simulink model "dc_motor_openloop_verification"  (R2026b)
settings: Solver=VariableStepAuto  StopTime=5.0
undefined symbols (not defined in the file): b, J, K, L, R
settings Model: Creator=nouran  LastModifiedBy=nouran

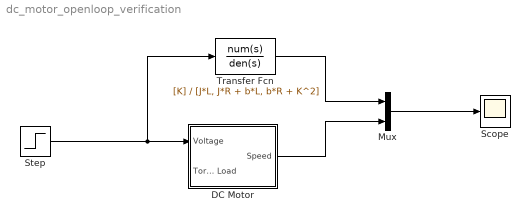
== system dc_motor_openloop_verification ==
  DC Motor : Subsystem
  Mux : Mux  Inputs=2
  Scope : Scope
      settings: ActiveDisplayYMinimum=0.00044834884289504662  ActiveDisplayYMaximum=0.11663294750657929
  Step : Step  Time=0  SampleTime=0
  Transfer Fcn : TransferFcn  Numerator=[K]  Denominator=[J*L, J*R + b*L, b*R + K^2]
  wires:
  Step/1 -> Transfer Fcn/1, DC Motor/1(Voltage)
  Mux/1 -> Scope/1
  Transfer Fcn/1 -> Mux/1
  DC Motor/1(Speed) -> Mux/2

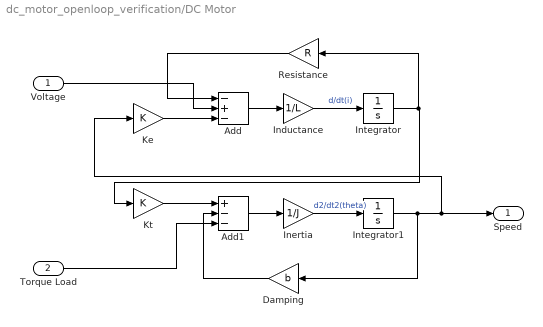
== system dc_motor_openloop_verification/DC Motor ==
  Voltage : Inport
  Torque Load : Inport  Port=2
  Add : Sum  Inputs=-+-
  Add1 : Sum  Inputs=+--
  Damping : Gain  Gain=b
  Inductance : Gain  Gain=1/L
  Inertia : Gain  Gain=1/J
  Integrator : Integrator
  Integrator1 : Integrator
  Ke : Gain  Gain=K
  Kt : Gain  Gain=K
  Resistance : Gain  Gain=R
  Speed : Outport
  wires:
  Resistance/1 -> Add/1
  Integrator/1 -> Resistance/1, Kt/1
  Add/1 -> Inductance/1
  Inductance/1 -> Integrator/1  "d/dt(i)"
  Voltage/1 -> Add/2
  Kt/1 -> Add1/1
  Ke/1 -> Add/3
  Add1/1 -> Inertia/1
  Integrator1/1 -> Speed/1, Ke/1, Damping/1
  Inertia/1 -> Integrator1/1  "d2/dt2(theta)"
  Damping/1 -> Add1/2
  Torque Load/1 -> Add1/3
